simulink model "LAB6_motor_control"  (R2026a)
settings: Solver=FixedStepAuto  FixedStep=0.001
undefined symbols (not defined in the file or in its folder): dspblkCoreblockFVToolHelper, gcbh
settings Model: Creator=ms110  LastModifiedBy=ms110

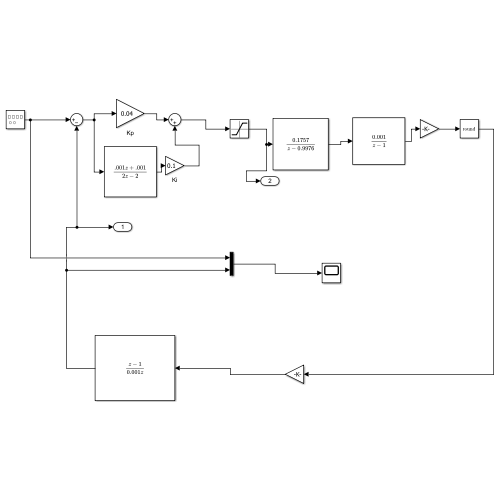
[thumbnail: Simulink's stored preview of the top-level diagram]
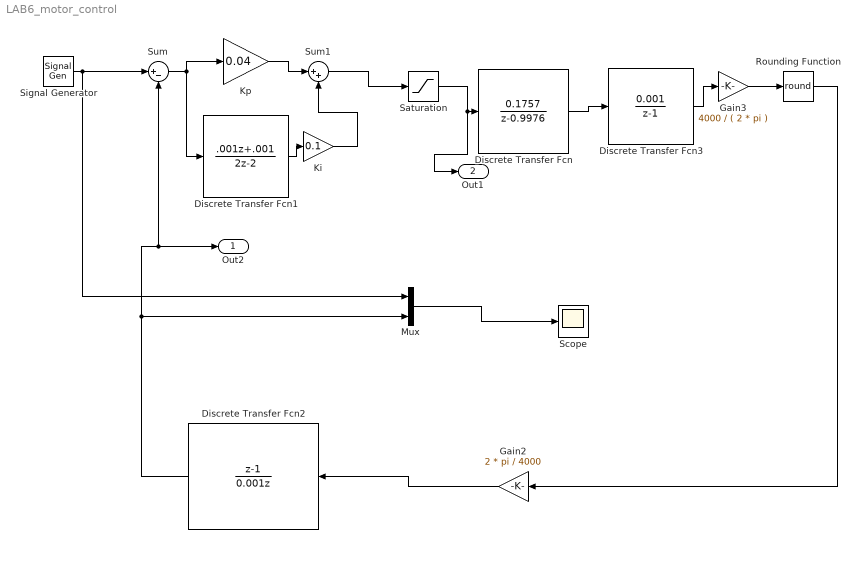
== system LAB6_motor_control ==
  Discrete Transfer Fcn : DiscreteTransferFcn  LoadFcn=dspblkCoreblockFVToolHelper(gcbh,'load');  Numerator=[0.1757]  Denominator=[1 -0.9976]
      settings: CopyFcn=dspblkCoreblockFVToolHelper(gcbh,'copy');  DeleteFcn=dspblkCoreblockFVToolHelper(gcbh,'close');  ModelCloseFcn=dspblkCoreblockFVToolHelper(gcbh,'close');  PreSaveFcn=dspblkCoreblockFVToolHelper(gcbh,'presave');  PostSaveFcn=dspblkCoreblockFVToolHelper(gcbh,'postsave');  CloseFcn=dspblkCoreblockFVToolHelper(gcbh,'close');
  Discrete Transfer Fcn1 : DiscreteTransferFcn  LoadFcn=dspblkCoreblockFVToolHelper(gcbh,'load');  Numerator=[.001 .001]  Denominator=[2 -2]
      settings: CopyFcn=dspblkCoreblockFVToolHelper(gcbh,'copy');  DeleteFcn=dspblkCoreblockFVToolHelper(gcbh,'close');  ModelCloseFcn=dspblkCoreblockFVToolHelper(gcbh,'close');  PreSaveFcn=dspblkCoreblockFVToolHelper(gcbh,'presave');  PostSaveFcn=dspblkCoreblockFVToolHelper(gcbh,'postsave');  CloseFcn=dspblkCoreblockFVToolHelper(gcbh,'close');
  Discrete Transfer Fcn2 : DiscreteTransferFcn  LoadFcn=dspblkCoreblockFVToolHelper(gcbh,'load');  Numerator=[1 -1]  Denominator=[0.001 0]
      settings: CopyFcn=dspblkCoreblockFVToolHelper(gcbh,'copy');  DeleteFcn=dspblkCoreblockFVToolHelper(gcbh,'close');  ModelCloseFcn=dspblkCoreblockFVToolHelper(gcbh,'close');  PreSaveFcn=dspblkCoreblockFVToolHelper(gcbh,'presave');  PostSaveFcn=dspblkCoreblockFVToolHelper(gcbh,'postsave');  CloseFcn=dspblkCoreblockFVToolHelper(gcbh,'close');
  Discrete Transfer Fcn3 : DiscreteTransferFcn  LoadFcn=dspblkCoreblockFVToolHelper(gcbh,'load');  Numerator=[0.001]  Denominator=[1 -1]
      settings: CopyFcn=dspblkCoreblockFVToolHelper(gcbh,'copy');  DeleteFcn=dspblkCoreblockFVToolHelper(gcbh,'close');  ModelCloseFcn=dspblkCoreblockFVToolHelper(gcbh,'close');  PreSaveFcn=dspblkCoreblockFVToolHelper(gcbh,'presave');  PostSaveFcn=dspblkCoreblockFVToolHelper(gcbh,'postsave');  CloseFcn=dspblkCoreblockFVToolHelper(gcbh,'close');
  Gain2 : Gain  Gain=2 * pi / 4000
  Gain3 : Gain  Gain=4000 / ( 2 * pi )
  Ki : Gain  Gain=0.1
  Kp : Gain  Gain=0.04
  Mux : Mux  Inputs=2
  Rounding Function : Rounding  Operator=round
  Saturation : Saturate  UpperLimit=10  LowerLimit=-10
  Scope : Scope
      settings: ActiveDisplayYMinimum=-117.56978952740837  ActiveDisplayYMaximum=120.0989002359311
  Signal Generator : SignalGenerator  WaveForm=square  Amplitude=100  Frequency=1/4
  Sum : Sum  Inputs=|+-
  Sum1 : Sum  Inputs=|++
  Out2 : Outport
  Out1 : Outport  Port=2
  wires:
  Sum/1 -> Discrete Transfer Fcn1/1, Kp/1
  Kp/1 -> Sum1/1
  Discrete Transfer Fcn1/1 -> Ki/1
  Ki/1 -> Sum1/2
  Sum1/1 -> Saturation/1
  Saturation/1 -> Out1/1, Discrete Transfer Fcn/1
  Discrete Transfer Fcn3/1 -> Gain3/1
  Gain3/1 -> Rounding Function/1
  Rounding Function/1 -> Gain2/1
  Gain2/1 -> Discrete Transfer Fcn2/1
  Discrete Transfer Fcn2/1 -> Out2/1, Sum/2, Mux/2
  Discrete Transfer Fcn/1 -> Discrete Transfer Fcn3/1
  Signal Generator/1 -> Mux/1, Sum/1
  Mux/1 -> Scope/1
